simulink model "VitalPlant"  (R2025b)
settings: Solver=ode4  StartTime=0  StopTime=1  FixedStep=dt  RelTol=1e-3
undefined symbols (not defined in the file): Ts, x0
settings Model: Creator=krish  LastModifiedBy=krish
settings DataIOCC: SaveFormat=StructureWithTime  SignalLogging=off
settings DebuggingCC: AlgebraicLoopMsg=error

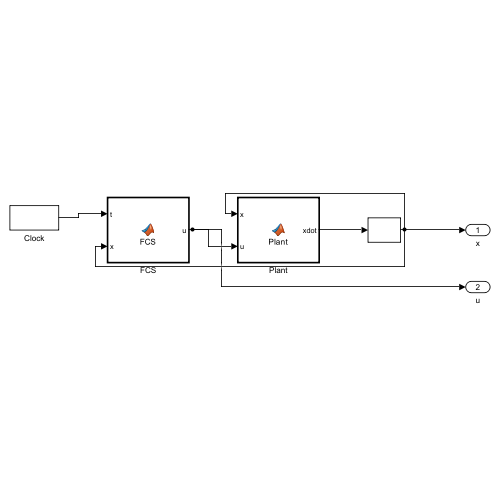
[thumbnail: Simulink's stored preview of the top-level diagram]
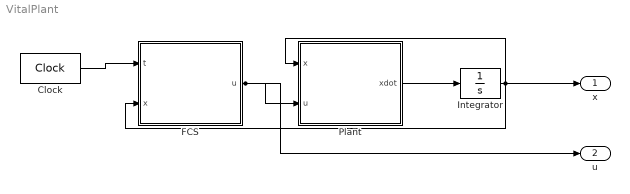
== system VitalPlant ==
  Clock : DigitalClock  SampleTime=Ts
  FCS : MATLAB Function  TreatAsAtomicUnit=on  SystemSampleTime=Ts
  Integrator : Integrator  InitialCondition=x0
  Plant : MATLAB Function  TreatAsAtomicUnit=on
  x : Outport
  u : Outport  Port=2
  wires:
  Clock/1 -> FCS/1(t)
  Integrator/1 -> FCS/2(x), Plant/1(x), x/1
  FCS/1(u) -> Plant/2(u), u/1
  Plant/1(xdot) -> Integrator/1

== matlab function VitalPlant/FCS ==
  data: t input; u output; x input
function u = FCS(t, x)
% GENERATED by vital.slx.build: the discrete FCS / input sample (zero-order held by Simulink).
coder.extrinsic('vital.slx.kernel');
u = zeros(4, 1);
u = vital.slx.kernel('fcs', t, x);

== matlab function VitalPlant/Plant ==
  data: x input; u input; xdot output
function xdot = Plant(x, u)
% GENERATED by vital.slx.build: the continuous plant (vital.plant.derivatives via vital.slx.kernel).
coder.extrinsic('vital.slx.kernel');
xdot = zeros(13, 1);
xdot = vital.slx.kernel('plant', x, u);
